simulink model "flightControlSystem"  (R2026b)
settings: Solver=ode3  StopTime=TFinal
PreLoadFcn:
  | InitVars;
undefined symbols (not defined in the file): control_power, feedforward_gains, integrator_limits, MC_PITCH_P, MC_PITCHRATE_D, MC_PITCHRATE_I, MC_PITCHRATE_MAX, MC_PITCHRATE_P, MC_ROLL_P, MC_ROLLRATE_D, MC_ROLLRATE_I, MC_ROLLRATE_MAX, MC_ROLLRATE_P, MC_YAW_P, MC_YAW_TQ_CUTOFF, MC_YAW_WEIGHT, MC_YAWRATE_D, MC_YAWRATE_I, MC_YAWRATE_MAX, MC_YAWRATE_P, MPC_ACC_DECOUPLE, MPC_LAND_ALT1, MPC_LAND_ALT2, MPC_LAND_ALT3, MPC_LAND_CRWL, MPC_LAND_SPEED, MPC_THR_HOVER, MPC_THR_MAX, MPC_THR_MIN, MPC_THR_XY_MARG, MPC_TILTMAX_AIR, MPC_VELD_LP, MPC_XY_P, MPC_XY_VEL_D_ACC, MPC_XY_VEL_I_ACC, MPC_XY_VEL_MAX, MPC_XY_VEL_P_ACC, MPC_Z_P, MPC_Z_VEL_D_ACC, MPC_Z_VEL_I_ACC, MPC_Z_VEL_MAX_DN, MPC_Z_VEL_MAX_UP, MPC_Z_VEL_P_ACC, SampleTime, timestamp
libraries: px4uORBlib x9, vrlib x8, aerolibutil x8, simulink x4, px4Utilslib x4, sharedutil x3, matrix_library x3, raspberrypiutilitieslib x2, px4Peripheralslib x2, sharedtransform x1, px4Sensorslib x1
(part 2 of 4)

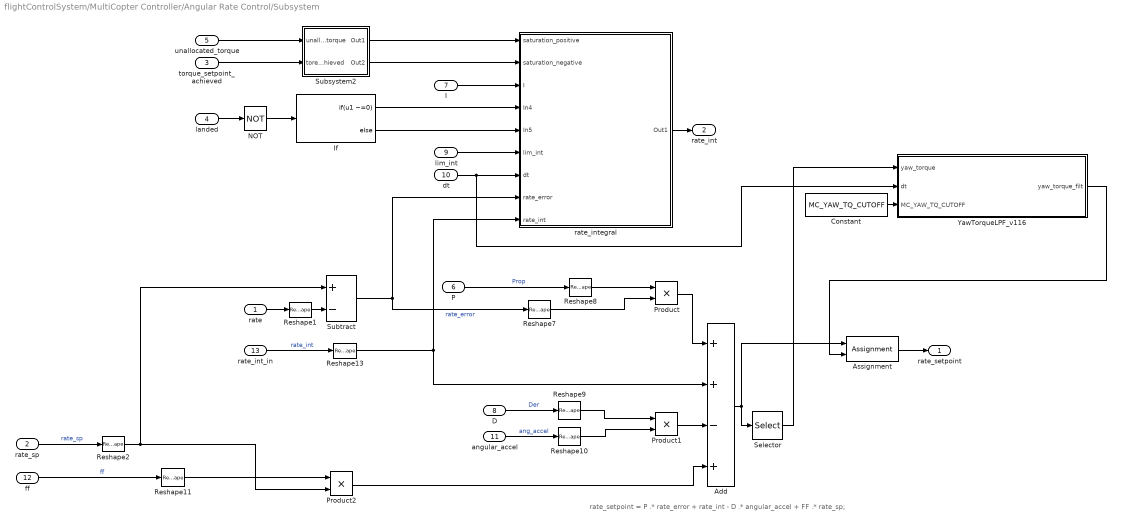
== system flightControlSystem/MultiCopter Controller/Angular Rate Control/Subsystem ==
  note: rate_setpoint = P .* rate_error + rate_int - D .* angular_accel + FF .* rate_sp;
  rate : Inport
  rate_sp : Inport  Port=2
  torque_setpoint_achieved : Inport  Port=3
  landed : Inport  Port=4
  unallocated_torque : Inport  Port=5
  P : Inport  Port=6
  I : Inport  Port=7
  D : Inport  Port=8
  lim_int : Inport  Port=9
  dt : Inport  Port=10
  angular_accel : Inport  Port=11
  ff : Inport  Port=12
  rate_int_in : Inport  Port=13
  Add : Sum  Inputs=++-+  AccumDataTypeStr=single
  Assignment : Assignment  DiagnosticForDimensions=Warning  IndexOptions=Index vector (dialog)  Indices=3  OutputSizes=1
  Constant : Constant  Value=MC_YAW_TQ_CUTOFF  SampleTime=-1
  If : If  IfExpression=u1 ~=0
  NOT : Logic  Operator=NOT  IconShape=distinctive  AllPortsSameDT=off  OutDataTypeStr=boolean
  Product : Product
  Product1 : Product
  Product2 : Product
  Reshape{1..2,7..11,13} (8 alike) : Reshape
  Selector : Selector  InputPortWidth=3  IndexOptions=Index vector (dialog)  Indices=3  OutputSizes=1
  Subsystem2 : Subsystem
  Subtract : Sum  Inputs=+-
  YawTorqueLPF_v116 : MATLAB Function  TreatAsAtomicUnit=on
  rate_integral : Subsystem
  rate_setpoint : Outport
  rate_int : Outport  Port=2
  wires:
  Reshape7/1 -> Product/2
  Reshape9/1 -> Product1/1
  ff/1 -> Reshape11/1  "ff"
  Product/1 -> Add/1
  landed/1 -> NOT/1
  rate_sp/1 -> Reshape2/1  "rate_sp"
  Subtract/1 -> Reshape7/1, rate_integral/8(rate_error)  "rate_error"
  NOT/1 -> If/1
  Reshape13/1 -> Add/2, rate_integral/9(rate_int)
  Reshape2/1 -> Subtract/1, Product2/2
  rate/1 -> Reshape1/1
  rate_int_in/1 -> Reshape13/1  "rate_int"
  Reshape11/1 -> Product2/1
  P/1 -> Reshape8/1  "Prop"
  D/1 -> Reshape9/1  "Der"
  angular_accel/1 -> Reshape10/1  "ang_accel"
  Product2/1 -> Add/4
  Reshape8/1 -> Product/1
  Reshape10/1 -> Product1/2
  Product1/1 -> Add/3
  Reshape1/1 -> Subtract/2
  unallocated_torque/1 -> Subsystem2/1(unallocated_torque)
  torque_setpoint_achieved/1 -> Subsystem2/2(torequ_sp_achieved)
  Subsystem2/1(Out1) -> rate_integral/1(saturation_positive)
  Subsystem2/2(Out2) -> rate_integral/2(saturation_negative)
  I/1 -> rate_integral/3(I)
  If/1 -> rate_integral/4(In4)
  If/2 -> rate_integral/5(In5)
  lim_int/1 -> rate_integral/6(lim_int)
  dt/1 -> YawTorqueLPF_v116/2(dt), rate_integral/7(dt)
  rate_integral/1(Out1) -> rate_int/1
  Add/1 -> Selector/1, Assignment/1
  Selector/1 -> YawTorqueLPF_v116/1(yaw_torque)
  YawTorqueLPF_v116/1(yaw_torque_filt) -> Assignment/2
  Constant/1 -> YawTorqueLPF_v116/3(MC_YAW_TQ_CUTOFF)
  Assignment/1 -> rate_setpoint/1

== system flightControlSystem/MultiCopter Controller/Angular Rate Control/get TargetGetAndSetpoint ==
  note: 1) Add Subsystem or Model blocks as valid variant choices.
      | 2) You cannot connect blocks at this level. At simulation, connectivity is automatically
      | determined, based on the active variant and port name matching.
  Control_Power : Inport
  Set target Position : Subsystem  VariantControl=Simulation == false
  Simulation Set target Position : Subsystem  VariantControl=Simulation == true

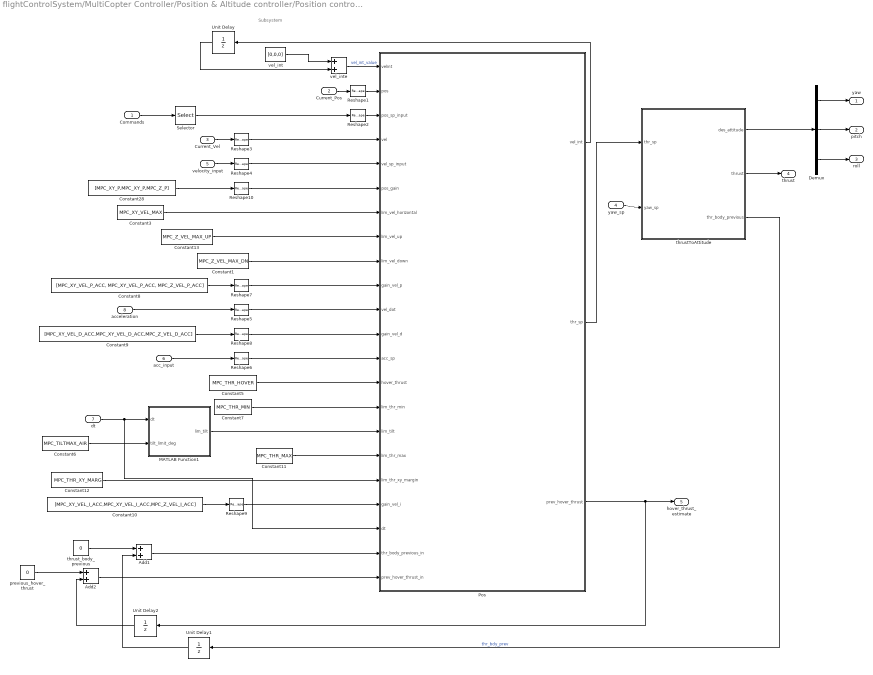
== system flightControlSystem/MultiCopter Controller/Position & Altitude controller/Position controller ==
  note: Subsystem
  Commands : Inport
  Current_Pos : Inport  Port=2
  Current_Vel : Inport  Port=3
  yaw_sp : Inport  Port=4
  velocity_input : Inport  Port=5
  acc_input : Inport  Port=6
  dt : Inport  Port=7
  acceleration : Inport  Port=8
  Add1 : Sum
  Add2 : Sum
  Constant1 : Constant  Value=MPC_Z_VEL_MAX_DN  OutDataTypeStr=single  SampleTime=-1
  Constant10 : Constant  Value=[MPC_XY_VEL_I_ACC,MPC_XY_VEL_I_ACC,MPC_Z_VEL_I_ACC]  OutDataTypeStr=single  SampleTime=-1
  Constant11 : Constant  Value=MPC_THR_MAX  OutDataTypeStr=single  SampleTime=-1
  Constant12 : Constant  Value=MPC_THR_XY_MARG  OutDataTypeStr=single  SampleTime=-1
  Constant13 : Constant  Value=MPC_Z_VEL_MAX_UP  OutDataTypeStr=single  SampleTime=-1
  Constant28 : Constant  Value=[MPC_XY_P,MPC_XY_P,MPC_Z_P]  OutDataTypeStr=single  SampleTime=-1
  Constant3 : Constant  Value=MPC_XY_VEL_MAX  OutDataTypeStr=single  SampleTime=-1
  Constant5 : Constant  Value=MPC_THR_HOVER  OutDataTypeStr=single  SampleTime=-1
  Constant6 : Constant  Value=MPC_TILTMAX_AIR  SampleTime=-1
  Constant7 : Constant  Value=MPC_THR_MIN  OutDataTypeStr=single  SampleTime=-1
  Constant8 : Constant  Value=[MPC_XY_VEL_P_ACC, MPC_XY_VEL_P_ACC, MPC_Z_VEL_P_ACC]  OutDataTypeStr=single  SampleTime=-1
  Constant9 : Constant  Value=[MPC_XY_VEL_D_ACC,MPC_XY_VEL_D_ACC,MPC_Z_VEL_D_ACC]  OutDataTypeStr=single  SampleTime=-1
  Demux : Demux  Outputs=3
  MATLAB Function1 : MATLAB Function  TreatAsAtomicUnit=on
  Pos : Subsystem
  Reshape{1..10} (10 alike) : Reshape
  Selector : Selector  InputPortWidth=4  IndexOptions=Index vector (dialog)  Indices=[1:3]  OutputSizes=1  RuntimeRangeChecks=off
  Unit Delay : UnitDelay  InitialCondition=[0; 0; 0]  SampleTime=-1
  Unit Delay1 : UnitDelay  SampleTime=-1
  Unit Delay2 : UnitDelay  SampleTime=-1
  previous_hover_thrust : Constant  Value=0  OutDataTypeStr=single  SampleTime=-1
  thrustToAttitude : Subsystem
  thrust_body_previous : Constant  Value=0  OutDataTypeStr=single  SampleTime=-1
  vel_int : Constant  Value=[0,0,0]  OutDataTypeStr=single  SampleTime=-1
  vel_inte : Sum
  yaw : Outport
  pitch : Outport  Port=2
  roll : Outport  Port=3
  thrust : Outport  Port=4
  hover_thrust_estimate : Outport  Port=5
  wires:
  thrustToAttitude/1(des_attitude) -> Demux/1
  previous_hover_thrust/1 -> Add2/1
  vel_int/1 -> vel_inte/1
  thrust_body_previous/1 -> Add1/1
  Commands/1 -> Selector/1
  Unit Delay1/1 -> Add1/2
  Constant6/1 -> MATLAB Function1/2(tilt_limit_deg)
  Unit Delay/1 -> vel_inte/2
  Unit Delay2/1 -> Add2/2
  Demux/1 -> yaw/1
  thrustToAttitude/2(thrust) -> thrust/1
  Pos/3(prev_hover_thrust) -> Unit Delay2/1, hover_thrust_estimate/1
  Pos/1(vel_int) -> Unit Delay/1
  Demux/3 -> roll/1
  Demux/2 -> pitch/1
  thrustToAttitude/3(thr_body_previous) -> Unit Delay1/1  "thr_bdy_prev"
  Pos/2(thr_sp) -> thrustToAttitude/1(thr_sp)
  Reshape9/1 -> Pos/19(gain_vel_i)
  Constant12/1 -> Pos/18(lim_thr_xy_margin)
  Constant11/1 -> Pos/17(lim_thr_max)
  dt/1 -> MATLAB Function1/1(dt), Pos/20(dt)
  Constant7/1 -> Pos/15(lim_thr_min)
  Constant5/1 -> Pos/14(hover_thrust)
  Reshape6/1 -> Pos/13(acc_sp)
  Reshape8/1 -> Pos/12(gain_vel_d)
  Reshape7/1 -> Pos/10(gain_vel_p)
  Constant13/1 -> Pos/8(lim_vel_up)
  Reshape10/1 -> Pos/6(pos_gain)
  Reshape4/1 -> Pos/5(vel_sp_input)
  Reshape5/1 -> Pos/11(vel_dot)
  Reshape3/1 -> Pos/4(vel)
  Reshape2/1 -> Pos/3(pos_sp_input)
  acc_input/1 -> Reshape6/1
  Constant3/1 -> Pos/7(lim_vel_horizontal)
  Constant8/1 -> Reshape7/1
  yaw_sp/1 -> thrustToAttitude/2(yaw_sp)
  Constant28/1 -> Reshape10/1
  Reshape1/1 -> Pos/2(pos)
  Constant1/1 -> Pos/9(lim_vel_down)
  acceleration/1 -> Reshape5/1
  velocity_input/1 -> Reshape4/1
  Current_Vel/1 -> Reshape3/1
  Selector/1 -> Reshape2/1
  Current_Pos/1 -> Reshape1/1
  Constant9/1 -> Reshape8/1
  Constant10/1 -> Reshape9/1
  MATLAB Function1/1(lim_tilt) -> Pos/16(lim_tilt)
  vel_inte/1 -> Pos/1(velint)  "vel_int_value"
  Add1/1 -> Pos/21(thr_body_previous_in)
  Add2/1 -> Pos/22(prev_hover_thrust_in)

== system flightControlSystem/get TargetGetAndSetpoint/Set target Position/Landing Logic ==
  Current_Pos : Inport
  land_trigger : Inport  Port=2
  MPC_LAND_ALT1_const : Constant  Value=MPC_LAND_ALT1  SampleTime=-1
  MPC_LAND_ALT2_const : Constant  Value=MPC_LAND_ALT2  SampleTime=-1
  MPC_LAND_ALT3_const : Constant  Value=MPC_LAND_ALT3  SampleTime=-1
  MPC_LAND_CRWL_const : Constant  Value=MPC_LAND_CRWL  SampleTime=-1
  MPC_LAND_SPEED_const : Constant  Value=MPC_LAND_SPEED  SampleTime=-1
  MPC_Z_VEL_MAX_DN_const : Constant  Value=MPC_Z_VEL_MAX_DN  SampleTime=-1
  PX4 Landing Logic : MATLAB Function  TreatAsAtomicUnit=on
  Selector1 : Selector  InputPortWidth=5  IndexOptions=Index vector (dialog)  Indices=[1:4]  OutputSizes=1  RuntimeRangeChecks=off
  pos_sp : Outport
  vel_sp : Outport  Port=2
  acc_sp : Outport  Port=3
  wires:
  Current_Pos/1 -> Selector1/1
  MPC_LAND_CRWL_const/1 -> PX4 Landing Logic/4(MPC_LAND_CRWL_in)
  Selector1/1 -> PX4 Landing Logic/2(states)
  MPC_LAND_SPEED_const/1 -> PX4 Landing Logic/3(MPC_LAND_SPEED_in)
  MPC_LAND_ALT1_const/1 -> PX4 Landing Logic/5(MPC_LAND_ALT1_in)
  MPC_Z_VEL_MAX_DN_const/1 -> PX4 Landing Logic/8(MPC_Z_VEL_MAX_DN_in)
  MPC_LAND_ALT2_const/1 -> PX4 Landing Logic/6(MPC_LAND_ALT2_in)
  MPC_LAND_ALT3_const/1 -> PX4 Landing Logic/7(MPC_LAND_ALT3_in)
  PX4 Landing Logic/1(pos_sp) -> pos_sp/1
  PX4 Landing Logic/2(vel_sp) -> vel_sp/1
  PX4 Landing Logic/3(acc_sp) -> acc_sp/1
  land_trigger/1 -> PX4 Landing Logic/1(land_trigger)

== system flightControlSystem/get TargetGetAndSetpoint/Set target Position/Logger ==
  DesiredPosition : Inport
  DesiredVelocity : Inport  Port=2
  DesiredAcceleration : Inport  Port=3
  States : Inport  Port=4
  Cast To Single{,1..13} (14 alike) : DataTypeConversion  OutDataTypeStr=single  SaturateOnIntegerOverflow=off  RndMeth=Floor
  Demux : Demux
  Demux1 : Demux
  Demux2 : Demux  Outputs=3
  Demux3 : Demux  Outputs=3
  PX4 ULog : px4Utilslib/PX4 ULog  Commented=on  uORBMsg=FlightChecks
  Rate Transition : RateTransition
  Rate Transition2 : RateTransition
  Selector : Selector  InputPortWidth=5  IndexOptions=Index vector (dialog)  Indices=[1:4]  OutputSizes=1
  wires:
  Cast To Single2/1 -> ?
  Demux/1 -> Cast To Single/1
  Cast To Single5/1 -> PX4 ULog/2
  Rate Transition2/1 -> Demux1/1
  Demux1/3 -> Cast To Single6/1
  Cast To Single7/1 -> PX4 ULog/4
  Demux1/1 -> Cast To Single4/1
  Rate Transition/1 -> Demux/1
  Cast To Single6/1 -> PX4 ULog/3
  DesiredPosition/1 -> Rate Transition2/1
  DesiredAcceleration/1 -> Demux3/1
  Demux1/2 -> Cast To Single5/1
  Demux2/1 -> Cast To Single8/1
  Cast To Single4/1 -> PX4 ULog/1
  Demux3/2 -> Cast To Single12/1
  Demux/2 -> Cast To Single1/1
  Demux1/4 -> Cast To Single7/1
  Cast To Single8/1 -> ?
  Demux2/2 -> Cast To Single9/1
  Cast To Single9/1 -> ?
  Cast To Single10/1 -> ?
  Demux2/3 -> Cast To Single10/1
  Demux3/1 -> Cast To Single11/1
  Cast To Single11/1 -> ?
  Cast To Single13/1 -> ?
  Cast To Single12/1 -> ?
  Demux3/3 -> Cast To Single13/1
  Cast To Single/1 -> ?
  Cast To Single1/1 -> ?
  Demux/3 -> Cast To Single2/1
  Demux/4 -> Cast To Single3/1
  Cast To Single3/1 -> ?
  States/1 -> Selector/1
  DesiredVelocity/1 -> Demux2/1
  Selector/1 -> Rate Transition/1

== system flightControlSystem/get TargetGetAndSetpoint/Set target Position/RC Failsafe Signal ==
  Constant1 : Constant  SampleTime=-1
  MATLAB Function : MATLAB Function  TreatAsAtomicUnit=on
  Radio Control Transmitter1 : px4Sensorslib/Radio Control Transmitter  channel1=off  channel2=off  channel3=off  channel4=off  channel5=off  channel6=off  channel7=off  channel8=on  channel_count=off  rssi=on  rc_input_source=off  timestamp_last_signal=off  time_stamp=off  sampleTime=1/250  BlockingMode=off  BlockTimeout=5
  Rate Transition3 : RateTransition
  Switch1 : Switch  Criteria=u2 ~= 0  SaturateOnIntegerOverflow=off  InputSameDT=off
  Unit Delay : UnitDelay  SampleTime=-1
  Land_Trigger : Outport
  wires:
  Constant1/1 -> Switch1/1
  Radio Control Transmitter1/3 -> MATLAB Function/3(RSSI)
  Radio Control Transmitter1/2 -> MATLAB Function/2(ch8)
  Radio Control Transmitter1/1 -> MATLAB Function/1(status)
  MATLAB Function/1(out) -> Rate Transition3/1
  Rate Transition3/1 -> Switch1/2
  Unit Delay/1 -> Switch1/3
  Switch1/1 -> Unit Delay/1, Land_Trigger/1

== system flightControlSystem/get TargetGetAndSetpoint/Set target Position/Setpoints Selector ==
  Land_Pos : Inport
  Land_Vel : Inport  Port=2
  Land_Acc : Inport  Port=3
  LandTrigger : Inport  Port=4
  Des_Pos : Inport  Port=5
  Des_Vel : Inport  Port=6
  Des_Acc : Inport  Port=7
  Acc Switch : Switch  Criteria=u2 > Threshold  SaturateOnIntegerOverflow=off  InputSameDT=off
  Rate Transition2 : RateTransition
  Rate Transition4 : RateTransition
  Rate Transition5 : RateTransition
  Reshape : Reshape
  Switch : Switch  Criteria=u2 > Threshold  SaturateOnIntegerOverflow=off  InputSameDT=off
  Vel Switch : Switch  Criteria=u2 > Threshold  SaturateOnIntegerOverflow=off  InputSameDT=off
  des_pos : Outport
  des_vel : Outport  Port=2
  des_acc : Outport  Port=3
  wires:
  Land_Acc/1 -> Acc Switch/1
  Acc Switch/1 -> Rate Transition5/1
  Reshape/1 -> Switch/1
  LandTrigger/1 -> Vel Switch/2, Switch/2, Acc Switch/2
  Switch/1 -> Rate Transition2/1
  Vel Switch/1 -> Rate Transition4/1
  Land_Pos/1 -> Reshape/1
  Land_Vel/1 -> Vel Switch/1
  Rate Transition2/1 -> des_pos/1
  Des_Pos/1 -> Switch/3
  Rate Transition4/1 -> des_vel/1
  Des_Vel/1 -> Vel Switch/3
  Rate Transition5/1 -> des_acc/1
  Des_Acc/1 -> Acc Switch/3

== system flightControlSystem/get TargetGetAndSetpoint/Set target Position/Setpoints from Perception Module ==
  CurrentPosition : Inport
  AND : Logic  IconShape=distinctive  AllPortsSameDT=off  OutDataTypeStr=boolean
  Cast To Boolean : DataTypeConversion  OutDataTypeStr=boolean  SaturateOnIntegerOverflow=off  RndMeth=Floor
  Cast To Double : DataTypeConversion  OutDataTypeStr=double  SaturateOnIntegerOverflow=off  RndMeth=Floor
  Compare To Constant1 : simulink/Logic and Bit Operations/Compare To Constant  relop===  const=222  OutDataTypeStr=boolean
  Demux : Demux  Outputs=11
  Enabled Subsystem : Subsystem  TreatAsAtomicUnit=on
  Mux : Mux
  Mux1 : Mux  Inputs=3
  Mux2 : Mux  Inputs=3
  Protocol Decoder : raspberrypiutilitieslib/Protocol Decoder  IsParseCSV=off  Header=[134]  FieldTable={ 'Field1', '11', 'single', 'Little endian' }  IsVariableSizeLastField=off  MaxVariableSizeFieldLength=[]  IsChecksumRequired=off  ChecksumAlgorithm=XOR of bytes  ChecksumSize=[]  TerminatorOption=<none>  CustomTerminatorVal=[]  IsInputLengthAvailable=off
  Selector : Selector  InputPortWidth=5  IndexOptions=Index vector (dialog)  Indices=[5]  OutputSizes=1  RuntimeRangeChecks=off
  Serial Receive : px4Peripheralslib/Serial Receive  SCIModule=/dev/ttyACM0  DataType=uint8  DataLength=45  OutputStatus=on  SampleTime=1/10  BlockingMode=off  PartialData=on  Timeout=5
  Switch2 : Switch  Criteria=u2 > Threshold  SaturateOnIntegerOverflow=off  InputSameDT=off
  Terminator : Terminator
  Terminator1 : Terminator
  Unit Delay : UnitDelay  SampleTime=-1
  des Position : Outport
  desired Velocity : Outport  Port=2
  desired Acceleration : Outport  Port=3
  wires:
  Demux/1 -> Mux/1
  Demux/3 -> Mux/3
  Demux/11 -> Compare To Constant1/1
  Mux2/1 -> desired Acceleration/1
  AND/1 -> Enabled Subsystem/Enable
  Demux/6 -> Mux1/2
  Demux/10 -> Mux2/3
  Selector/1 -> Cast To Boolean/1
  Compare To Constant1/1 -> AND/2, Switch2/2
  Protocol Decoder/1 -> Cast To Double/1
  Cast To Double/1 -> Demux/1
  Demux/2 -> Mux/2
  Mux1/1 -> desired Velocity/1
  Demux/9 -> Mux2/2
  Protocol Decoder/2 -> Terminator/1
  Cast To Boolean/1 -> AND/1
  Demux/8 -> Mux2/1
  Demux/5 -> Mux1/1
  Serial Receive/1 -> Protocol Decoder/1
  Mux/1 -> Switch2/1
  Unit Delay/1 -> Switch2/3
  Switch2/1 -> des Position/1, Unit Delay/1
  CurrentPosition/1 -> Selector/1, Enabled Subsystem/1(CurrentPosition)
  Demux/4 -> Mux/4
  Demux/7 -> Mux1/3
  Serial Receive/2 -> Terminator1/1

== system flightControlSystem/get TargetGetAndSetpoint/Simulation Set target Position/Landing Logic ==
  Current_Pos : Inport
  land_trigger : Inport  Port=2
  MPC_LAND_ALT1_const : Constant  Value=MPC_LAND_ALT1  SampleTime=-1
  MPC_LAND_ALT2_const : Constant  Value=MPC_LAND_ALT2  SampleTime=-1
  MPC_LAND_ALT3_const : Constant  Value=MPC_LAND_ALT3  SampleTime=-1
  MPC_LAND_CRWL_const : Constant  Value=MPC_LAND_CRWL  SampleTime=-1
  MPC_LAND_SPEED_const : Constant  Value=MPC_LAND_SPEED  SampleTime=-1
  MPC_Z_VEL_MAX_DN_const : Constant  Value=MPC_Z_VEL_MAX_DN  SampleTime=-1
  PX4 Landing Logic : MATLAB Function  TreatAsAtomicUnit=on
  Selector1 : Selector  InputPortWidth=5  IndexOptions=Index vector (dialog)  Indices=[1:4]  OutputSizes=1  RuntimeRangeChecks=off
  pos_sp : Outport
  vel_sp : Outport  Port=2
  acc_sp : Outport  Port=3
  wires:
  Current_Pos/1 -> Selector1/1
  MPC_LAND_CRWL_const/1 -> PX4 Landing Logic/4(MPC_LAND_CRWL_in)
  Selector1/1 -> PX4 Landing Logic/2(states)
  MPC_LAND_SPEED_const/1 -> PX4 Landing Logic/3(MPC_LAND_SPEED_in)
  MPC_LAND_ALT1_const/1 -> PX4 Landing Logic/5(MPC_LAND_ALT1_in)
  MPC_Z_VEL_MAX_DN_const/1 -> PX4 Landing Logic/8(MPC_Z_VEL_MAX_DN_in)
  MPC_LAND_ALT2_const/1 -> PX4 Landing Logic/6(MPC_LAND_ALT2_in)
  MPC_LAND_ALT3_const/1 -> PX4 Landing Logic/7(MPC_LAND_ALT3_in)
  PX4 Landing Logic/1(pos_sp) -> pos_sp/1
  PX4 Landing Logic/2(vel_sp) -> vel_sp/1
  PX4 Landing Logic/3(acc_sp) -> acc_sp/1
  land_trigger/1 -> PX4 Landing Logic/1(land_trigger)

== system flightControlSystem/get TargetGetAndSetpoint/Simulation Set target Position/Setpoints Selector ==
  Land_Pos : Inport
  Land_Vel : Inport  Port=2
  Land_Acc : Inport  Port=3
  LandTrigger : Inport  Port=4
  Des_Pos : Inport  Port=5
  Des_Vel : Inport  Port=6
  Des_Acc : Inport  Port=7
  Acc Switch : Switch  Criteria=u2 > Threshold  SaturateOnIntegerOverflow=off  InputSameDT=off
  Rate Transition2 : RateTransition
  Rate Transition4 : RateTransition
  Rate Transition5 : RateTransition
  Reshape : Reshape
  Switch : Switch  Criteria=u2 > Threshold  SaturateOnIntegerOverflow=off  InputSameDT=off
  Vel Switch : Switch  Criteria=u2 > Threshold  SaturateOnIntegerOverflow=off  InputSameDT=off
  des_pos : Outport
  des_vel : Outport  Port=2
  des_acc : Outport  Port=3
  wires:
  Land_Acc/1 -> Acc Switch/1
  Acc Switch/1 -> Rate Transition5/1
  Reshape/1 -> Switch/1
  LandTrigger/1 -> Vel Switch/2, Switch/2, Acc Switch/2
  Switch/1 -> Rate Transition2/1
  Vel Switch/1 -> Rate Transition4/1
  Land_Pos/1 -> Reshape/1
  Land_Vel/1 -> Vel Switch/1
  Rate Transition2/1 -> des_pos/1
  Des_Pos/1 -> Switch/3
  Rate Transition4/1 -> des_vel/1
  Des_Vel/1 -> Vel Switch/3
  Rate Transition5/1 -> des_acc/1
  Des_Acc/1 -> Acc Switch/3

== system flightControlSystem/Actuator Commands/Simulation Actuator Commands/Mixer/Battery_Scaling ==
  In1 : Inport
  In2 : Inport  Port=2
  Compare To Constant : simulink/Logic and Bit Operations/Compare To Constant  relop=~=  const=0  OutDataTypeStr=boolean
  Constant : Constant  SampleTime=SampleTime
  Demux1 : Demux  Outputs=3
  Gain : Gain  Gain=-1
  Product : Product
  Product2 : Product
  Saturation1 : Saturate  UpperLimit=1  LowerLimit=-1
  Saturation2 : Saturate  UpperLimit=1  LowerLimit=-1
  Switch : Switch  Criteria=u2 > Threshold  SaturateOnIntegerOverflow=off  InputSameDT=off
  Switch1 : Switch  Criteria=u2 > Threshold  SaturateOnIntegerOverflow=off  InputSameDT=off
  thrust_setpoint : Outport
  pitch : Outport  Port=2
  roll : Outport  Port=3
  yaw : Outport  Port=4
  wires:
  Constant/1 -> Product2/2, Compare To Constant/1, Product/2  "<scale>"
  In1/1 -> Switch/3, Product/1
  In2/1 -> Switch1/3, Product2/1
  Switch/1 -> Gain/1
  Product/1 -> Switch/1
  Gain/1 -> Saturation2/1
  Demux1/3 -> yaw/1
  Switch1/1 -> Saturation1/1
  Compare To Constant/1 -> Switch1/2, Switch/2
  Saturation1/1 -> Demux1/1  "torque_setpoint"
  Product2/1 -> Switch1/1
  Demux1/1 -> roll/1
  Demux1/2 -> pitch/1
  Saturation2/1 -> thrust_setpoint/1  "thrust_setpoint"

== system flightControlSystem/MultiCopter Controller/Angle_Control/AttitudeControl/vectorToQuaternion ==
  src : Inport
  dst : Inport  Port=2
  AND : Logic  Commented=on  IconShape=distinctive  AllPortsSameDT=off  OutDataTypeStr=boolean
  Abs : Abs  Commented=on  SaturateOnIntegerOverflow=off
  Cast To Double : DataTypeConversion  OutDataTypeStr=double  SaturateOnIntegerOverflow=off  RndMeth=Floor
  Constant : Constant  Commented=on  Value=0  SampleTime=-1
  Cross Product : matrix_library/Cross Product  Commented=on
  Dot Product : DotProduct  Commented=on  OutDataTypeStr=Inherit: Inherit via internal rule
  MATLAB Function : MATLAB Function  TreatAsAtomicUnit=on
  Normalize Vector : vrlib/Utilities/Normalize Vector  maxzero=0
  Relational Operator : RelationalOperator  Commented=on  Operator=<  OutDataTypeStr=boolean  RndMeth=Simplest  InputSameDT=off
  Relational Operator1 : RelationalOperator  Commented=on  Operator=<  OutDataTypeStr=boolean  RndMeth=Simplest  InputSameDT=off
  Switch : Switch  Commented=on  Criteria=u2 > Threshold  SaturateOnIntegerOverflow=off  InputSameDT=off
  eps : Constant  Value=1e-5  SampleTime=-1
  norm : MATLAB Function  Commented=on  TreatAsAtomicUnit=on
  quat : Outport
  wires:
  src/1 -> Abs/1, MATLAB Function/1(src), Dot Product/1, Cross Product/1
  dst/1 -> MATLAB Function/2(dst), Dot Product/2, Cross Product/2
  Cross Product/1 -> norm/1(u)
  norm/1(y) -> Relational Operator/1
  eps/1 -> Relational Operator/2
  Relational Operator/1 -> AND/1
  Dot Product/1 -> Relational Operator1/1
  Constant/1 -> Relational Operator1/2
  Relational Operator1/1 -> AND/2
  AND/1 -> Switch/2
  MATLAB Function/1(q) -> Cast To Double/1
  Normalize Vector/1 -> quat/1
  Cast To Double/1 -> Normalize Vector/1

== system flightControlSystem/MultiCopter Controller/Angular Rate Control/Subsystem/Subsystem2 ==
  unallocated_torque : Inport
  torequ_sp_achieved : Inport  Port=2
  If Action Subsystem1 : Subsystem  TreatAsAtomicUnit=on
  If1 : If  IfExpression=u1 ~= 0
  Merge1 : Merge
  Merge2 : Merge
  NOT1 : Logic  Operator=NOT  IconShape=distinctive  AllPortsSameDT=off  OutDataTypeStr=boolean
  Subsystem1 : Subsystem
  Out1 : Outport
  Out2 : Outport  Port=2
  wires:
  If Action Subsystem1/2(saturation_negative) -> Merge2/2
  Merge1/1 -> Out1/1
  If Action Subsystem1/1(saturation_positive) -> Merge1/2
  If1/2 -> If Action Subsystem1/Action
  Subsystem1/2(saturation_negative) -> Merge2/1
  If1/1 -> Subsystem1/Action
  NOT1/1 -> If1/1
  Subsystem1/1(saturation_positive) -> Merge1/1
  torequ_sp_achieved/1 -> NOT1/1
  unallocated_torque/1 -> Subsystem1/1(unallocated_torque)
  Merge2/1 -> Out2/1

== system flightControlSystem/MultiCopter Controller/Angular Rate Control/Subsystem/rate_integral ==
  saturation_positive : Inport
  saturation_negative : Inport  Port=2
  I : Inport  Port=3
  In4 : Inport  Port=4
  In5 : Inport  Port=5
  lim_int : Inport  Port=6
  dt : Inport  Port=7
  rate_error : Inport  Port=8
  rate_int : Inport  Port=9
  If Action Subsystem : Subsystem  TreatAsAtomicUnit=on
  Merge : Merge
  Subsystem : Subsystem
  Out1 : Outport
  wires:
  If Action Subsystem/1(Out1) -> Merge/2
  saturation_positive/1 -> Subsystem/1(saturation_positive)
  In4/1 -> Subsystem/Action
  lim_int/1 -> Subsystem/4(lim_int)
  dt/1 -> Subsystem/7(dt)
  Subsystem/1(out_rateInt) -> Merge/1
  saturation_negative/1 -> Subsystem/2(saturation_negative)
  rate_int/1 -> Subsystem/6(rate_int), If Action Subsystem/1(rate_int_in)
  Merge/1 -> Out1/1
  I/1 -> Subsystem/3(I)
  rate_error/1 -> Subsystem/5(rate_error)
  In5/1 -> If Action Subsystem/Action

== system flightControlSystem/MultiCopter Controller/Angular Rate Control/get TargetGetAndSetpoint/Set target Position ==
  Control_Power : Inport
  Bus Assignment : BusAssignment  AssignedSignals=timestamp,control_power
  PX4 Timestamp : px4Utilslib/PX4 Timestamp  SampleTime=-1
  PX4 uORB Message : px4uORBlib/PX4 uORB Message  uORBMsg=ActuatorControlsStatus  uORBTopicName=actuator_controls_status_0  isSingleTopicMsg=off  SampleTime=-1
  PX4 uORB Write : px4uORBlib/PX4 uORB Write  uORBMsg=ActuatorControlsStatus  uORBTopicName=actuator_controls_status_0  PublishOption=None  OutputPublishedInstanceNum=off  selectInstanceNum=1  OutputStatus=off  isSingleTopicMsg=off
  wires:
  PX4 Timestamp/1 -> Bus Assignment/2
  PX4 uORB Message/1 -> Bus Assignment/1
  Bus Assignment/1 -> PX4 uORB Write/1
  Control_Power/1 -> Bus Assignment/3

== system flightControlSystem/MultiCopter Controller/Angular Rate Control/get TargetGetAndSetpoint/Simulation Set target Position ==
  Control_Power : Inport
  Terminator3 : Terminator
  wires:
  Control_Power/1 -> Terminator3/1

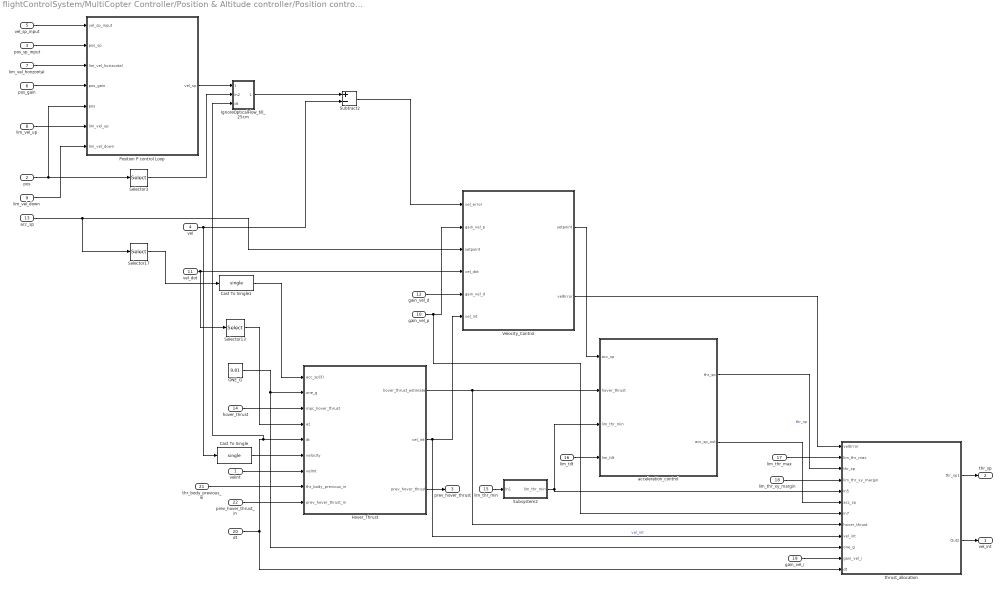
== system flightControlSystem/MultiCopter Controller/Position & Altitude controller/Position controller/Pos ==
  velint : Inport
  pos : Inport  Port=2
  pos_sp_input : Inport  Port=3
  vel : Inport  Port=4
  vel_sp_input : Inport  Port=5
  pos_gain : Inport  Port=6
  lim_vel_horizontal : Inport  Port=7
  lim_vel_up : Inport  Port=8
  lim_vel_down : Inport  Port=9
  gain_vel_p : Inport  Port=10
  vel_dot : Inport  Port=11
  gain_vel_d : Inport  Port=12
  acc_sp : Inport  Port=13
  hover_thrust : Inport  Port=14
  lim_thr_min : Inport  Port=15
  lim_tilt : Inport  Port=16
  lim_thr_max : Inport  Port=17
  lim_thr_xy_margin : Inport  Port=18
  gain_vel_i : Inport  Port=19
  dt : Inport  Port=20
  thr_body_previous_in : Inport  Port=21
  prev_hover_thrust_in : Inport  Port=22
  Cast To Single : DataTypeConversion  OutDataTypeStr=single  SaturateOnIntegerOverflow=off  RndMeth=Floor
  Cast To Single1 : DataTypeConversion  OutDataTypeStr=single  SaturateOnIntegerOverflow=off  RndMeth=Floor
  Hover_Thrust : Subsystem
  IgnoreOpticalFlow_till_25cm : Subsystem
  ONE_G : Constant  Value=9.81  OutDataTypeStr=single  SampleTime=-1
  Position P control Loop : Subsystem
  Selector13 : Selector  InputPortWidth=3  IndexOptions=Index vector (dialog)  Indices=3  OutputSizes=1  RuntimeRangeChecks=off
  Selector17 : Selector  InputPortWidth=3  IndexOptions=Index vector (dialog)  Indices=3  OutputSizes=1  RuntimeRangeChecks=off
  Selector3 : Selector  InputPortWidth=3  IndexOptions=Index vector (dialog)  Indices=[3]  OutputSizes=1  RuntimeRangeChecks=off
  Subsystem2 : Subsystem
  Subtract2 : Sum  Inputs=+-
  Velocity_Control : Subsystem
  acceleration_control : Subsystem
  thrust_allocation : Subsystem
  vel_int : Outport
  thr_sp : Outport  Port=2
  prev_hover_thrust : Outport  Port=3
  wires:
  acc_sp/1 -> Velocity_Control/3("setpoint "), Selector17/1
  vel_sp_input/1 -> Position P control Loop/1(vel_sp_input)
  pos_sp_input/1 -> Position P control Loop/2(pos_sp)
  pos/1 -> Selector3/1, Position P control Loop/5(pos)
  lim_vel_horizontal/1 -> Position P control Loop/3(lim_vel_horizontal)
  pos_gain/1 -> Position P control Loop/4(pos_gain)
  lim_vel_up/1 -> Position P control Loop/6(lim_vel_up)
  lim_vel_down/1 -> Position P control Loop/7(lim_vel_down)
  Position P control Loop/1(vel_sp) -> IgnoreOpticalFlow_till_25cm/1(vel_so)
  vel_dot/1 -> Velocity_Control/4(vel_dot), Selector13/1
  Selector3/1 -> IgnoreOpticalFlow_till_25cm/2(In2)
  vel/1 -> Cast To Single/1, Subtract2/2
  Selector17/1 -> Cast To Single1/1
  IgnoreOpticalFlow_till_25cm/1(Out1) -> Subtract2/1
  Cast To Single1/1 -> Hover_Thrust/1(acc_sp(3))
  hover_thrust/1 -> Hover_Thrust/3(mpc_hover_thrust)
  Selector13/1 -> Hover_Thrust/4(az)
  ONE_G/1 -> thrust_allocation/10(one_g), Hover_Thrust/2(one_g)
  Cast To Single/1 -> Hover_Thrust/6(velocity)
  velint/1 -> Hover_Thrust/7(velInt)
  dt/1 -> IgnoreOpticalFlow_till_25cm/3(dt), Hover_Thrust/5(dt), thrust_allocation/12(dt)
  thr_body_previous_in/1 -> Hover_Thrust/8(thr_body_previous_in)
  prev_hover_thrust_in/1 -> Hover_Thrust/9(prev_hover_thrust_in)
  Subtract2/1 -> Velocity_Control/1(vel_error)
  gain_vel_d/1 -> Velocity_Control/5(gain_vel_d)
  gain_vel_p/1 -> thrust_allocation/7(In7), Velocity_Control/2(gain_vel_p)
  lim_thr_min/1 -> Subsystem2/1(In1)
  thrust_allocation/1(thr_sp1) -> thr_sp/1
  lim_tilt/1 -> acceleration_control/4(lim_tilt)
  Hover_Thrust/2(vel_int) -> thrust_allocation/9(vel_int), Velocity_Control/6(vel_int)  "vel_int"
  Hover_Thrust/1(hover_thrust_estimate) -> thrust_allocation/8(hover_thrust), acceleration_control/2(hover_thrust)
  Hover_Thrust/3(prev_hover_thrust) -> prev_hover_thrust/1
  Velocity_Control/2(velError) -> thrust_allocation/1(velError)
  Velocity_Control/1(setpoint) -> acceleration_control/1(acc_sp)
  Subsystem2/1(lim_thr_min) -> acceleration_control/3(lim_thr_min), thrust_allocation/5(In5)
  lim_thr_max/1 -> thrust_allocation/2(lim_thr_max)
  lim_thr_xy_margin/1 -> thrust_allocation/4(lim_thr_xy_margin)
  acceleration_control/2(acc_sp_out) -> thrust_allocation/6(acc_sp)
  acceleration_control/1(thr_sp) -> thrust_allocation/3(thr_sp)  "thr_sp"
  gain_vel_i/1 -> thrust_allocation/11(gain_vel_i)
  thrust_allocation/2(Out2) -> vel_int/1

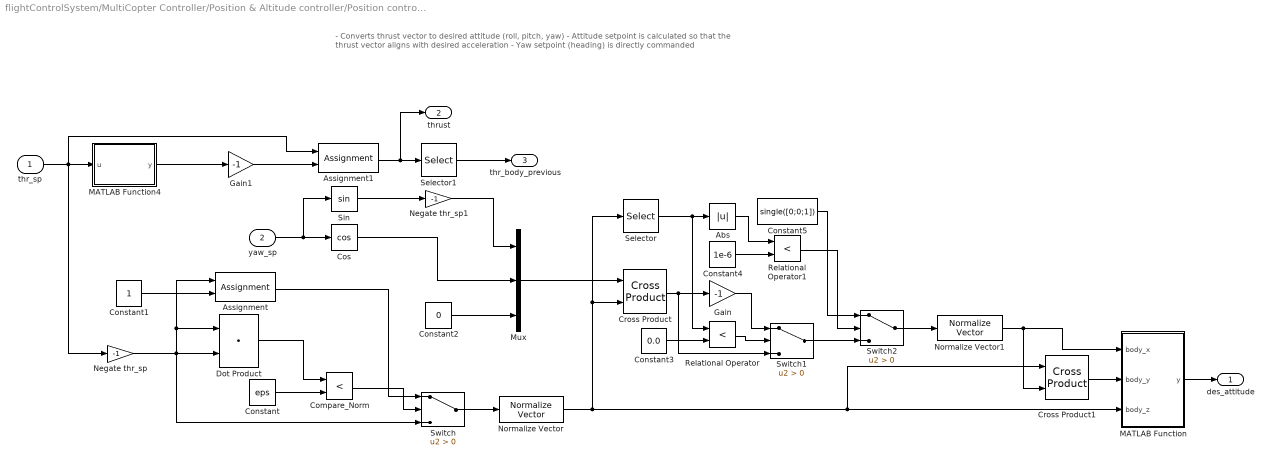
== system flightControlSystem/MultiCopter Controller/Position & Altitude controller/Position controller/thrustToAttitude ==
  note: - Converts thrust vector to desired attitude (roll, pitch, yaw)
      | - Attitude setpoint is calculated so that the thrust vector aligns with desired acceleration
      | - Yaw setpoint (heading) is directly commanded
  thr_sp : Inport
  yaw_sp : Inport  Port=2
  Abs : Abs  SaturateOnIntegerOverflow=off
  Assignment : Assignment  DiagnosticForDimensions=Warning  IndexOptions=Index vector (dialog)  Indices=[3]  OutputSizes=1  RuntimeRangeChecks=off
  Assignment1 : Assignment  DiagnosticForDimensions=Warning  IndexOptions=Index vector (dialog)  Indices=3  OutputSizes=1  RuntimeRangeChecks=off
  Compare_Norm : RelationalOperator  Operator=<  OutDataTypeStr=boolean  RndMeth=Simplest  InputSameDT=off
  Constant : Constant  Value=eps  SampleTime=-1
  Constant1 : Constant  SampleTime=-1
  Constant2 : Constant  Value=0  SampleTime=-1
  Constant3 : Constant  Value=0.0  SampleTime=-1
  Constant4 : Constant  Value=1e-6  OutDataTypeStr=single  SampleTime=-1
  Constant5 : Constant  Value=single([0;0;1])  OutDataTypeStr=single  SampleTime=-1
  Cos : Trigonometry  Operator=cos
  Cross Product : matrix_library/Cross Product
  Cross Product1 : matrix_library/Cross Product
  Dot Product : DotProduct  OutDataTypeStr=Inherit: Inherit via internal rule
  Gain : Gain  Gain=-1
  Gain1 : Gain  Gain=-1
  MATLAB Function : MATLAB Function  TreatAsAtomicUnit=on
  MATLAB Function4 : MATLAB Function  TreatAsAtomicUnit=on
  Mux : Mux  Inputs=3
  Negate thr_sp : Gain  Gain=-1
  Negate thr_sp1 : Gain  Gain=-1
  Normalize Vector : vrlib/Utilities/Normalize Vector  maxzero=0
  Normalize Vector1 : vrlib/Utilities/Normalize Vector  maxzero=0
  Relational Operator : RelationalOperator  Operator=<  OutDataTypeStr=boolean  RndMeth=Simplest  InputSameDT=off
  Relational Operator1 : RelationalOperator  Operator=<  OutDataTypeStr=boolean  RndMeth=Simplest  InputSameDT=off
  Selector : Selector  InputPortWidth=3  IndexOptions=Index vector (dialog)  Indices=3  OutputSizes=1  RuntimeRangeChecks=off
  Selector1 : Selector  InputPortWidth=3  IndexOptions=Index vector (dialog)  Indices=3  OutputSizes=1  RuntimeRangeChecks=off
  Sin : Trigonometry
  Switch : Switch  Criteria=u2 > Threshold  SaturateOnIntegerOverflow=off  InputSameDT=off
  Switch1 : Switch  Criteria=u2 > Threshold  SaturateOnIntegerOverflow=off  InputSameDT=off
  Switch2 : Switch  Criteria=u2 > Threshold  SaturateOnIntegerOverflow=off  InputSameDT=off
  des_attitude : Outport
  thrust : Outport  Port=2
  thr_body_previous : Outport  Port=3
  wires:
  Switch2/1 -> Normalize Vector1/1
  Gain/1 -> Switch1/1
  Gain1/1 -> Assignment1/2
  Negate thr_sp1/1 -> Mux/1
  thr_sp/1 -> Assignment1/1, MATLAB Function4/1(u), Negate thr_sp/1
  Constant/1 -> Compare_Norm/2
  Constant1/1 -> Assignment/2
  Selector1/1 -> thr_body_previous/1
  Sin/1 -> Negate thr_sp1/1
  MATLAB Function4/1(y) -> Gain1/1
  Dot Product/1 -> Compare_Norm/1
  yaw_sp/1 -> Cos/1, Sin/1
  Negate thr_sp/1 -> Dot Product/2, Switch/3, Assignment/1, Dot Product/1
  Assignment/1 -> Switch/1
  Assignment1/1 -> Selector1/1, thrust/1
  Cos/1 -> Mux/2
  Compare_Norm/1 -> Switch/2
  Constant3/1 -> Relational Operator/2
  Constant2/1 -> Mux/3
  Switch/1 -> Normalize Vector/1
  Mux/1 -> Cross Product/1
  Normalize Vector/1 -> Cross Product1/1, MATLAB Function/3(body_z), Selector/1, Cross Product/2
  Selector/1 -> Abs/1, Relational Operator/1
  Cross Product/1 -> Switch1/3, Gain/1
  Abs/1 -> Relational Operator1/1
  Relational Operator1/1 -> Switch2/2
  Constant5/1 -> Switch2/1
  Constant4/1 -> Relational Operator1/2
  Relational Operator/1 -> Switch1/2
  Switch1/1 -> Switch2/3
  Normalize Vector1/1 -> MATLAB Function/1(body_x), Cross Product1/2
  Cross Product1/1 -> MATLAB Function/2(body_y)
  MATLAB Function/1(y) -> des_attitude/1

== system flightControlSystem/get TargetGetAndSetpoint/Set target Position/Setpoints from Perception Module/Enabled Subsystem ==
  CurrentPosition : Inport
  Enable : EnablePort
  Cast To Single : DataTypeConversion  OutDataTypeStr=single  SaturateOnIntegerOverflow=off  RndMeth=Floor
  Constant : Constant  Value=221  OutDataTypeStr=single  SampleTime=-1
  Demux : Demux
  Protocol Encoder : raspberrypiutilitieslib/Protocol Encoder  Header=[123]  FieldTable={ 'Field1', '1', 'single', 'Little endian'; 'Field2', '1', 'single', 'Little endian'; 'Field3', '1', 'single', 'Little endian'; 'Field4', '1', 'single', 'Little endian'; 'Field5', '1', 'single', 'Little endian' }  IsChecksumRequired=off  ChecksumAlgorithm=XOR of bytes  ChecksumSize=[]  TerminatorOption=<none>  CustomTerminatorVal=[]
  Selector : Selector  InputPortWidth=5  IndexOptions=Index vector (dialog)  Indices=[1:4]  OutputSizes=1  RuntimeRangeChecks=off
  Serial Transmit : px4Peripheralslib/Serial Transmit  SCIModule=/dev/ttyACM0
  wires:
  CurrentPosition/1 -> Selector/1
  Cast To Single/1 -> Demux/1
  Constant/1 -> Protocol Encoder/5
  Selector/1 -> Cast To Single/1
  Demux/1 -> Protocol Encoder/1
  Demux/2 -> Protocol Encoder/2
  Demux/3 -> Protocol Encoder/3
  Demux/4 -> Protocol Encoder/4
  Protocol Encoder/1 -> Serial Transmit/1

== system flightControlSystem/MultiCopter Controller/Angular Rate Control/Subsystem/Subsystem2/If Action Subsystem1 ==
  Action Port : ActionPort  ActionPortLabel=else
  Constant1 : Constant  Value=[0, 0, 0]  OutDataTypeStr=boolean  SampleTime=-1
  Constant2 : Constant  Value=[0, 0, 0]  OutDataTypeStr=boolean  SampleTime=-1
  saturation_positive : Outport
  saturation_negative : Outport  Port=2
  wires:
  Constant2/1 -> saturation_positive/1
  Constant1/1 -> saturation_negative/1

== system flightControlSystem/MultiCopter Controller/Angular Rate Control/Subsystem/Subsystem2/Subsystem1 ==
  unallocated_torque : Inport
  Action Port : ActionPort  ActionPortLabel=if(u1 ~= 0)
  Constant1 : Constant  Value=eps  SampleTime=-1
  Constant3 : Constant  Value=-eps  SampleTime=-1
  Relational Operator1 : RelationalOperator  Operator=>  OutDataTypeStr=boolean  RndMeth=Simplest  InputSameDT=off
  Relational Operator2 : RelationalOperator  Operator=<  OutDataTypeStr=boolean  RndMeth=Simplest  InputSameDT=off
  saturation_positive : Outport
  saturation_negative : Outport  Port=2
  wires:
  Relational Operator2/1 -> saturation_negative/1
  Constant1/1 -> Relational Operator1/2
  unallocated_torque/1 -> Relational Operator2/1, Relational Operator1/1
  Constant3/1 -> Relational Operator2/2
  Relational Operator1/1 -> saturation_positive/1

== system flightControlSystem/MultiCopter Controller/Angular Rate Control/Subsystem/rate_integral/If Action Subsystem ==
  rate_int_in : Inport
  Action Port : ActionPort  ActionPortLabel=else
  Out1 : Outport
  wires:
  rate_int_in/1 -> Out1/1

== system flightControlSystem/MultiCopter Controller/Angular Rate Control/Subsystem/rate_integral/Subsystem ==
  saturation_positive : Inport
  saturation_negative : Inport  Port=2
  I : Inport  Port=3
  lim_int : Inport  Port=4
  rate_error : Inport  Port=5
  rate_int : Inport  Port=6
  dt : Inport  Port=7
  Action Port : ActionPort  ActionPortLabel=if(u1 ~=0)
  Update_Integral : Subsystem  TreatAsAtomicUnit=on
  out_rateInt : Outport
  wires:
  rate_error/1 -> Update_Integral/5(rate_error)
  saturation_positive/1 -> Update_Integral/1(satPos)
  rate_int/1 -> Update_Integral/6(rate_int)
  saturation_negative/1 -> Update_Integral/2(saNeg)
  I/1 -> Update_Integral/3(I)
  dt/1 -> Update_Integral/7(dt)
  lim_int/1 -> Update_Integral/4(lim_int)
  Update_Integral/1(out_rateInt) -> out_rateInt/1

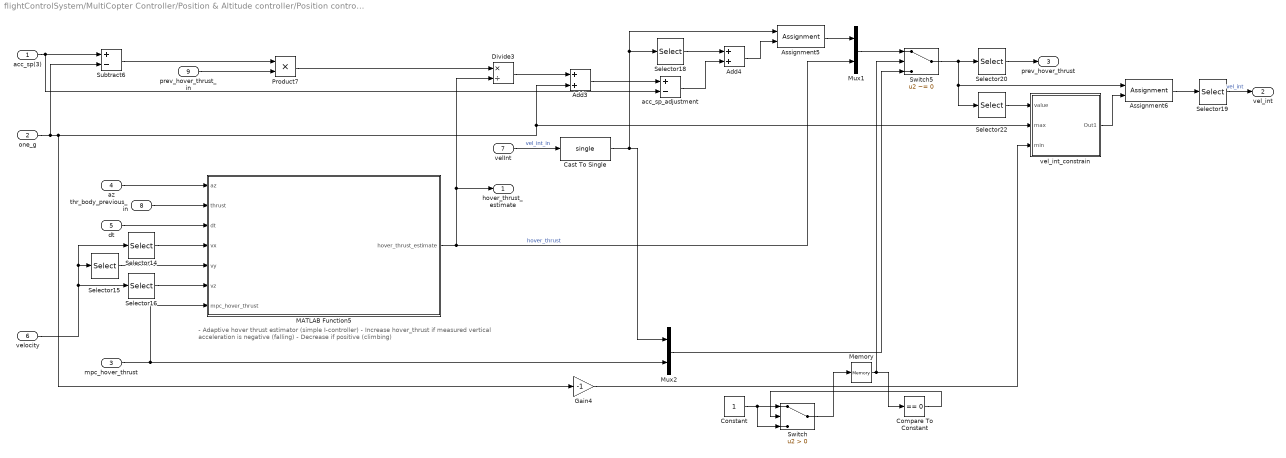
== system flightControlSystem/MultiCopter Controller/Position & Altitude controller/Position controller/Pos/Hover_Thrust ==
  note: - Adaptive hover thrust estimator (simple I-controller)
      | - Increase hover_thrust if measured vertical acceleration is negative (falling)
      | - Decrease if positive (climbing)
  acc_sp(3) : Inport
  one_g : Inport  Port=2
  mpc_hover_thrust : Inport  Port=3
  az : Inport  Port=4
  dt : Inport  Port=5
  velocity : Inport  Port=6
  velInt : Inport  Port=7
  thr_body_previous_in : Inport  Port=8
  prev_hover_thrust_in : Inport  Port=9
  Add3 : Sum
  Add4 : Sum
  Assignment5 : Assignment  DiagnosticForDimensions=Warning  IndexOptions=Index vector (dialog)  Indices=3  OutputSizes=1  RuntimeRangeChecks=off
  Assignment6 : Assignment  DiagnosticForDimensions=Warning  IndexOptions=Index vector (dialog)  Indices=3  OutputSizes=1  RuntimeRangeChecks=off
  Cast To Single : DataTypeConversion  OutDataTypeStr=single  SaturateOnIntegerOverflow=off  RndMeth=Floor
  Compare To Constant : simulink/Logic and Bit Operations/Compare To Constant  relop===  const=0  OutDataTypeStr=boolean
  Constant : Constant  SampleTime=-1
  Divide3 : Product  Inputs=*/
  Gain4 : Gain  Gain=-1
  MATLAB Function5 : MATLAB Function  TreatAsAtomicUnit=on
  Memory : Memory  InheritSampleTime=on
  Mux1 : Mux  Inputs=2
  Mux2 : Mux  Inputs=2
  Product7 : Product
  Selector14 : Selector  InputPortWidth=3  IndexOptions=Index vector (dialog)  Indices=[1]  OutputSizes=1  RuntimeRangeChecks=off
  Selector15 : Selector  InputPortWidth=3  IndexOptions=Index vector (dialog)  Indices=2  OutputSizes=1  RuntimeRangeChecks=off
  Selector16 : Selector  InputPortWidth=3  IndexOptions=Index vector (dialog)  Indices=3  OutputSizes=1  RuntimeRangeChecks=off
  Selector18 : Selector  InputPortWidth=3  IndexOptions=Index vector (dialog)  Indices=3  OutputSizes=1  RuntimeRangeChecks=off
  Selector19 : Selector  InputPortWidth=4  IndexOptions=Index vector (dialog)  Indices=[1 2 3]  OutputSizes=1  RuntimeRangeChecks=off
  Selector20 : Selector  InputPortWidth=4  IndexOptions=Index vector (dialog)  Indices=4  OutputSizes=1  RuntimeRangeChecks=off
  Selector22 : Selector  InputPortWidth=4  IndexOptions=Index vector (dialog)  Indices=3  OutputSizes=1  RuntimeRangeChecks=off
  Subtract6 : Sum  Inputs=+-
  Switch : Switch  Criteria=u2 > Threshold  SaturateOnIntegerOverflow=off  InputSameDT=off
  Switch5 : Switch  Criteria=u2 ~= 0  SaturateOnIntegerOverflow=off  InputSameDT=off
  acc_sp_adjustment : Sum  Inputs=+-
  vel_int_constrain : Subsystem
  hover_thrust_estimate : Outport
  vel_int : Outport  Port=2
  prev_hover_thrust : Outport  Port=3
  wires:
  Constant/1 -> Switch/3, Switch/1
  dt/1 -> MATLAB Function5/3(dt)
  prev_hover_thrust_in/1 -> Product7/2
  acc_sp(3)/1 -> acc_sp_adjustment/2, Subtract6/1
  Compare To Constant/1 -> Switch/2
  az/1 -> MATLAB Function5/1(az)
  thr_body_previous_in/1 -> MATLAB Function5/2(thrust)
  velocity/1 -> Selector15/1, Selector14/1, Selector16/1
  one_g/1 -> Add3/2, vel_int_constrain/2(max), Gain4/1, Subtract6/2
  Subtract6/1 -> Product7/1
  Switch5/1 -> Assignment6/1, Selector22/1, Selector20/1
  Selector14/1 -> MATLAB Function5/4(vx)
  Selector15/1 -> MATLAB Function5/5(vy)
  Selector16/1 -> MATLAB Function5/6(vz)
  mpc_hover_thrust/1 -> Mux2/2, MATLAB Function5/7(mpc_hover_thrust)
  Product7/1 -> Divide3/1
  Add4/1 -> Assignment5/2
  MATLAB Function5/1(hover_thrust_estimate) -> Divide3/2, hover_thrust_estimate/1, Mux1/2  "hover_thrust"
  velInt/1 -> Cast To Single/1  "vel_int_in"
  Divide3/1 -> Add3/1
  Add3/1 -> acc_sp_adjustment/1
  Cast To Single/1 -> Assignment5/1, Selector18/1, Mux2/1
  Gain4/1 -> vel_int_constrain/3(min)
  vel_int_constrain/1(Out1) -> Assignment6/2
  Selector18/1 -> Add4/1
  acc_sp_adjustment/1 -> Add4/2
  Mux2/1 -> Switch5/3
  Assignment5/1 -> Mux1/1
  Switch/1 -> Memory/1
  Mux1/1 -> Switch5/1
  Memory/1 -> Switch5/2, Compare To Constant/1
  Selector20/1 -> prev_hover_thrust/1
  Selector22/1 -> vel_int_constrain/1(value)
  Assignment6/1 -> Selector19/1
  Selector19/1 -> vel_int/1  "vel_int"

== system flightControlSystem/MultiCopter Controller/Position & Altitude controller/Position controller/Pos/IgnoreOpticalFlow_till_25cm ==
  note: Keep Velocity X,Y = 0 till drone reaches 25 cm height to avoid reacting to Optical flow noise
  vel_so : Inport
  In2 : Inport  Port=2
  dt : Inport  Port=3
  Assignment : Assignment  DiagnosticForDimensions=Warning  IndexOptions=Index vector (dialog)  Indices=[1,2]  OutputSizes=1  RuntimeRangeChecks=off
  Assignment1 : Assignment  DiagnosticForDimensions=Warning  IndexOptions=Index vector (dialog)  Indices=3  OutputSizes=1
  Constant : Constant  Value=-0.25  SampleTime=-1
  Constant1 : Constant  Value=0  SampleTime=-1
  MATLAB Function : MATLAB Function  TreatAsAtomicUnit=on
  Relational Operator : RelationalOperator  Operator=>  OutDataTypeStr=boolean  RndMeth=Simplest  InputSameDT=off
  Selector : Selector  InputPortWidth=3  IndexOptions=Index vector (dialog)  Indices=[3]  OutputSizes=1
  Switch : Switch  Criteria=u2 > Threshold  SaturateOnIntegerOverflow=off  InputSameDT=off
  Out1 : Outport
  wires:
  vel_so/1 -> Switch/3, Assignment/1, Selector/1
  Relational Operator/1 -> Switch/2
  Constant1/1 -> Assignment/2
  Assignment/1 -> Switch/1
  In2/1 -> Relational Operator/1
  Constant/1 -> Relational Operator/2
  Selector/1 -> MATLAB Function/1(vel_sp_z)
  MATLAB Function/1(vel_sp_z_limited) -> Assignment1/2
  Assignment1/1 -> Out1/1
  Switch/1 -> Assignment1/1
  dt/1 -> MATLAB Function/2(dt)

== system flightControlSystem/MultiCopter Controller/Position & Altitude controller/Position controller/Pos/Position P control Loop ==
  note: - Computes position error: pos_error = pos_sp_input - pos
      | - Generates velocity setpoint from position error using
      | proportional gain:
      | vel_sp_position = pos_gain .* pos_error
  vel_sp_input : Inport
  pos_sp : Inport  Port=2
  lim_vel_horizontal : Inport  Port=3
  pos_gain : Inport  Port=4
  pos : Inport  Port=5
  lim_vel_up : Inport  Port=6
  lim_vel_down : Inport  Port=7
  Gain : Gain  Gain=-1
  Mux : Mux  Inputs=2
  Product : Product
  Selector : Selector  InputPortWidth=3  IndexOptions=Index vector (dialog)  Indices=[1 2]  OutputSizes=1  RuntimeRangeChecks=off
  Selector1 : Selector  InputPortWidth=3  IndexOptions=Index vector (dialog)  Indices=[1 2]  OutputSizes=1  RuntimeRangeChecks=off
  Selector2 : Selector  InputPortWidth=3  IndexOptions=Index vector (dialog)  Indices=[3]  OutputSizes=1  RuntimeRangeChecks=off
  Subsystem : Subsystem
  Subtract : Sum  Inputs=+-
  Subtract1 : Sum  Inputs=+-
  constrain : Subsystem
  constrained_xy : Subsystem
  vel_sp : Outport
  wires:
  pos_sp/1 -> Subtract/1
  pos/1 -> Subtract/2
  Subtract/1 -> Product/1  "pos_error"
  pos_gain/1 -> Product/2
  constrained_xy/1(Out1) -> Mux/1
  lim_vel_up/1 -> Gain/1
  Selector/1 -> Subtract1/2, constrained_xy/1(v0)
  constrain/1(Out1) -> Mux/2
  Selector1/1 -> Subtract1/1
  Selector2/1 -> constrain/1(value)
  Gain/1 -> constrain/2(min)
  lim_vel_down/1 -> constrain/3(max)
  Subtract1/1 -> constrained_xy/2(v1)
  lim_vel_horizontal/1 -> constrained_xy/3(max_val)
  Mux/1 -> vel_sp/1
  Subsystem/2(setpoint) -> Selector2/1, Selector1/1
  vel_sp_input/1 -> Subsystem/1("setpoint ")
  Product/1 -> Subsystem/2(addition)
  Subsystem/1(vector) -> Selector/1

== system flightControlSystem/MultiCopter Controller/Position & Altitude controller/Position controller/Pos/Subsystem2 ==
  In1 : Inport
  Constant : Constant  Value=10e-4  SampleTime=-1
  Max : MinMax  Function=max  Inputs=2
  lim_thr_min : Outport
  wires:
  In1/1 -> Max/1
  Constant/1 -> Max/2
  Max/1 -> lim_thr_min/1

== system flightControlSystem/MultiCopter Controller/Position & Altitude controller/Position controller/Pos/Velocity_Control ==
  vel_error : Inport
  gain_vel_p : Inport  Port=2
  "setpoint " : Inport  Port=3
  vel_dot : Inport  Port=4
  gain_vel_d : Inport  Port=5
  vel_int : Inport  Port=6
  Add : Sum  Inputs=++-
  MATLAB Function2 : MATLAB Function  TreatAsAtomicUnit=on
  Product1 : Product
  Product2 : Product
  setpoint : Outport
  velError : Outport  Port=2
  wires:
  gain_vel_p/1 -> Product1/2
  vel_error/1 -> velError/1, Product1/1
  vel_dot/1 -> Product2/1
  "setpoint "/1 -> MATLAB Function2/1("setpoint ")
  gain_vel_d/1 -> Product2/2
  vel_int/1 -> Add/2
  Product1/1 -> Add/1
  Product2/1 -> Add/3
  Add/1 -> MATLAB Function2/2(addition)
  MATLAB Function2/1(setpoint) -> setpoint/1

== system flightControlSystem/MultiCopter Controller/Position & Altitude controller/Position controller/Pos/acceleration_control ==
  note: Converts acceleration setpoint to thrust vector, applies tilt and thrust constraints
  acc_sp : Inport
  hover_thrust : Inport  Port=2
  lim_thr_min : Inport  Port=3
  lim_tilt : Inport  Port=4
  ACC_Decoupling : Subsystem
  Constant1 : Constant  Value=[0;0;1]  SampleTime=-1
  Constant2 : Constant  Value=9.81  SampleTime=-1
  Constant3 : Constant  Value=[0;0;1]  SampleTime=-1
  Divide : Product  Inputs=*/
  Divide1 : Product  Inputs=*/
  Dot Product : DotProduct  OutDataTypeStr=Inherit: Inherit via internal rule
  Gain : Gain  Gain=-1
  Gain1 : Gain  Gain=-1  OutDataTypeStr=double
  Gain2 : Gain  Gain=-1  OutDataTypeStr=double
  Min : MinMax  Inputs=2
  Mux : Mux  Inputs=3
  Normalize Vector : vrlib/Utilities/Normalize Vector  maxzero=0
  Product : Product
  Product1 : Product
  Selector : Selector  InputPortWidth=3  IndexOptions=Index vector (dialog)  Indices=1  OutputSizes=1  RuntimeRangeChecks=off
  Selector1 : Selector  InputPortWidth=3  IndexOptions=Index vector (dialog)  Indices=2  OutputSizes=1  RuntimeRangeChecks=off
  Selector2 : Selector  InputPortWidth=3  IndexOptions=Index vector (dialog)  Indices=[3]  OutputSizes=1  RuntimeRangeChecks=off
  Subtract : Sum  Inputs=+-
  limitTilt : Subsystem
  thr_sp : Outport
  acc_sp_out : Outport  Port=2
  wires:
  lim_thr_min/1 -> Gain/1
  Selector/1 -> Gain1/1
  Constant2/1 -> Divide/2
  Gain1/1 -> Mux/1
  acc_sp/1 -> Selector/1, Selector2/1, Selector1/1, acc_sp_out/1
  Divide/1 -> Product/2
  hover_thrust/1 -> Subtract/2, Divide/1
  Selector2/1 -> ACC_Decoupling/1(In2), Product/1
  Selector1/1 -> Gain2/1
  Product/1 -> Subtract/1
  Gain2/1 -> Mux/2
  Subtract/1 -> Divide1/1
  Mux/1 -> Normalize Vector/1
  Normalize Vector/1 -> limitTilt/1(body_unit)
  Constant1/1 -> limitTilt/2(world_unit)
  Min/1 -> Product1/2
  lim_tilt/1 -> limitTilt/3(max_angle)
  limitTilt/1(Out1) -> Product1/1, Dot Product/2
  Constant3/1 -> Dot Product/1
  Dot Product/1 -> Divide1/2
  Divide1/1 -> Min/1
  Gain/1 -> Min/2
  Product1/1 -> thr_sp/1
  ACC_Decoupling/1(Out1) -> Mux/3
